simulink model "single_phase_dab"  (R2026b)
settings: Solver=ode23tb  StopTime=param.sim.simlength  FixedStep=param.glb_time.tc  MaxStep=param.glb_time.tc
values from neighbouring files (symbols this model uses):
  param = struct()    [init_model.m]
libraries: fl_lib x22, nesl_utility x15, discrete_time_low_pass_filter x7, lithium_ion_battery x2, pi_ctrl x2, full_bridge_ideal_switch x2, full_bridge_mosfet_based_with_thermal_model x2, full_bridge_mosfet_based_with_thermal_model_zvs x2, dab_single_phase_pwm_modulator x1, single_phase_transformer x1
(part 1 of 2)
settings Model: Creator=LTNBDA  LastModifiedBy=d.bagnara
settings SolverCC: AutoInsertRateTranBlk=on  SolverResetMethod=Robust  ZeroCrossAlgorithm=Adaptive  ZeroCrossControl=EnableAll
settings DataIOCC: DSMLogging=off  LimitDataPoints=on  MaxDataPoints=1  ReturnWorkspaceOutputs=off  SaveFormat=Array  SaveOutput=off  SaveTime=off  SignalLogging=off  SignalLoggingSaveFormat=ModelDataLogs
settings OptimizationCC: EfficientMapNaN2IntZero=off  LifeSpan=inf  MemsetInitFltsAndDblsToZero=off
settings DebuggingCC: ArithmeticOperatorsInVariantConditions=warning  FcnCallInpInsideContextMsg=warning  MergeDetectMultiDrivingBlocksExec=none  MultiTaskCondExecSysMsg=none  MultiTaskDSMMsg=warning  MultiTaskRateTransMsg=warning  SFNoUnconditionalDefaultTransitionDiag=warning  SFUnexpectedBacktrackingDiag=warning  SaveWithParameterizedLinksMsg=none  SignalResolutionControl=TryResolveAllWithWarning  SolverPrmCheckMsg=warning  StateNameClashWarn=warning
settings HardwareCC: ProdEndianess=Unspecified  ProdEqTarget=off  ProdHWDeviceType=Generic->64-bit Embedded Processor (LP64)  ProdIntDivRoundTo=Undefined  ProdLargestAtomicFloat=None  TargetEndianess=LittleEndian  TargetHWDeviceType=MATLAB Host  TargetIntDivRoundTo=Zero  TargetLongLongMode=on
settings ModelReferenceCC: PropagateSignalLabelsOutOfModel=off
settings SFSimCC: CustomCodeUndefinedFunction=UseInterfaceOnly  SimUseLocalCustomCode=off
settings SFSimCC: SimCustomHeaderCode=|
  | #include "rpi.h"
  | #include "rpi_simulink.h"
  | #include "mavgflt.h"
  | #include "mavgflt_simulink.h"
  | #include "mavgflts.h"
  | #include "mavgflts_simulink.h"
  | #include "dsmavgflt.h"
  | #include "dsmavgflt_simulink.h"
  | #include "bemf_obsv.h"
  | #include "bemf_obsv_simulink.h"
  | #include "bemf_obsv_load_est.h"
  | #include "bemf_obsv_load_est_simulink.h"
  | #include "dqvector_pi.h"
  | #include "dqvector_pi_simulink.h"
  | #include "sv_pwm_simulink.h"
  | #include "sv_pwm.h"
  | #include "first_harmonic_tracker.h"
  | #include "first_harmonic_tracker_simulink.h"
  | #include "dqpll_thyr.h"
  | #include "dqpll_thyr_simulink.h"
  | #include "dqpll_grid.h"
  | #include "dqpll_grid_simulink.h"
  | #include "linear_double_integrator_observer_simulink.h"
  | #include "linear_double_integrator_observer.h"
  | #include "sv_pwm_cm_simulink.h"
  | #include "sv_pwm_cm.h"
settings SFSimCC: SimUserIncludeDirs=|
  | include
  | src
settings SFSimCC: SimUserSources=|
  | "rpi.c"
  | "rpi_simulink.c"
  | "mavgflt_simulink.c"
  | "mavgflt.c"
  | "mavgflts_simulink.c"
  | "mavgflts.c"
  | "dsmavgflt_simulink.c"
  | "dsmavgflt.c"
  | "bemf_obsv_simulink.c"
  | "bemf_obsv.c"
  | "bemf_obsv_load_est_simulink.c"
  | "bemf_obsv_load_est.c"
  | "dqvector_pi.c"
  | "dqvector_pi_simulink.c"
  | "sv_pwm_simulink.c"
  | "sv_pwm.c"
  | "first_harmonic_tracker_simulink.c"
  | "first_harmonic_tracker.c"
  | "dqpll_thyr_simulink.c"
  | "dqpll_thyr.c"
  | "dqpll_grid_simulink.c"
  | "dqpll_grid.c"
  | "linear_double_integrator_observer_simulink.c"
  | "linear_double_integrator_observer.c"
  | "sv_pwm_cm_simulink.c"
  | "sv_pwm_cm.c"
settings RTWCC: CustomInclude=ccaller  RTWUseLocalCustomCode=off
settings CodeAppCC: StateflowObjectComments=on
settings GRTTargetCC: CombineOutputUpdateFcns=off  GRTInterface=on  TargetLangStandard=C89/C90 (ANSI)
settings ConfigComp: CovExternalEMLEnable=off  CovSaveCumulativeToWorkspaceVar=on  CovSaveSingleToWorkspaceVar=on
settings SimscapeCC: SimscapeNormalizeSystem=off  SimscapeUseEnergyAccounting=off

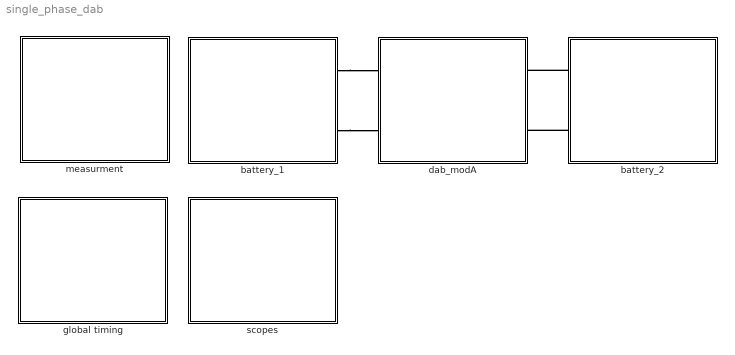
== system single_phase_dab ==
  battery_1 : Subsystem
  battery_2 : Subsystem
  dab_modA : Subsystem
  global timing : Subsystem
  measurment : Subsystem
  scopes : Subsystem
  connections:
  battery_2/RConn2 -- dab_modA/RConn2
  battery_2/RConn1 -- dab_modA/RConn1
  battery_1/RConn1 -- dab_modA/LConn1
  battery_1/RConn2 -- dab_modA/LConn2

== system single_phase_dab/battery_1 ==
  Electrical Reference1 : fl_lib/Electrical/Electrical Elements/Electrical Reference
  Solver Configuration : nesl_utility/Solver Configuration  PhysicalDomain=network_engine_domain  SubClassName=solver  LeftPortType=input  RightPortType=generic  Tones=[]  Harmonics=[]  SimulateNoise=off  Profile=off  UseLocalSampling=off  EnableSwitchedLinearOptims=on  FrequencyDomain=off  UseCCode=off  RelTol=0.001  AbsTol=0.001  MinStep=1e-09  ToWorkspace=off  RevertToSquareIcSolve=off  NumHomotopyIterations=100  PhasorMode=off  PhasorModeNumHarmonics=1  ConsistencySolver=NEWTON_FTOL  CanonicalOrdering=UNORDERED  OptimizeIntermediates=UNOPTIMIZED  MulticoreSolverChoice=BACKWARD_EULER  IndexReductionMethod=DerivativeReplacement  DoDC=off  ResidualTolerance=1e-09  ConsistencyTolSource=GLOBAL  ConsistencyAbsTol=0.001  ConsistencyRelTol=0.001  ConsistencyTolFactor=0.001  UseLocalSolver=on  LocalSolverChoice=NE_BACKWARD_EULER_ADVANCER  ResolveIndetEquations=on  FunctionEvalNumThread=1  LocalSolverSampleTime=param.glb_time.tc  DoFixedCost=on  MaxNonlinIter=param.sim.nonlinear_iterations  MaxModeIter=2  ComputeImpulses=off  ImpulseIterations=2  LinearAlgebra=auto  LinearAlgebraNumThread=0  EquationFormulation=NE_TIME_EF  DelaysMemoryBudget=1024  AutomaticFiltering=on  FilteringTimeConstant=0.001  PartitionStorageMethod=AS_NEEDED  PartitionMemoryBudget=1024  PartitionMethod=BALANCED  MultibodyUseLocalSolver=off  MultibodyLocalSolverChoice=ODE1  MultibodyLocalSolverSampleTime=0.001
  litium ion battery 1 : Scope
      settings: ActiveDisplayYMinimum=-166.63080014270002  ActiveDisplayYMaximum=1499.6922306374129  DataLoggingVariableName=ScopeData3
  litium_ion_battery : lithium_ion_battery/lithium_ion_battery  Q=param.battery.pack_1.Q  number_of_cells=param.battery.pack_1.number_of_cells  E_1=param.battery.pack_1.E_1  E0=param.battery.pack_1.E0  E1=param.battery.pack_1.E1  E2=param.battery.pack_1.E2  E3=param.battery.pack_1.E3  Elog=param.battery.pack_1.Elog  R0=param.battery.pack_1.R0  R1=param.battery.pack_1.R1  C1=param.battery.pack_1.C1  M=param.battery.pack_1.M  alpha=param.battery.pack_1.alpha  soc_init=param.battery.pack_1.soc_init  ts_battery=param.glb_time.ts_dab  q1Kalman=param.battery.pack_1.q1Kalman  q2Kalman=param.battery.pack_1.q2Kalman  q3Kalman=param.battery.pack_1.q3Kalman  rKalman=param.battery.pack_1.rKalman  tc=param.glb_time.tc  enable_white_noise_m=0  battery_voltage_init_m=param.battery.ocv_1
  single_phase_ui_measure : Subsystem
  dc+ : PMIOPort  Side=Right
  dc- : PMIOPort  Port=2  Side=Right
  wires:
  litium_ion_battery/1 -> litium ion battery 1/1
  connections:
  single_phase_ui_measure/LConn2 -- litium_ion_battery/RConn2 -- Electrical Reference1/LConn1 -- Solver Configuration/RConn1
  single_phase_ui_measure/RConn1 -- dc+/RConn1
  litium_ion_battery/RConn1 -- single_phase_ui_measure/LConn1
  dc-/RConn1 -- single_phase_ui_measure/RConn2

== system single_phase_dab/battery_2 ==
  Electrical Reference1 : fl_lib/Electrical/Electrical Elements/Electrical Reference
  litium ion battery 2 : Scope
      settings: ActiveDisplayYMinimum=-4779.68523514888  ActiveDisplayYMaximum=38953.418417165572  DataLoggingVariableName=ScopeData3
  litium_ion_battery : lithium_ion_battery/lithium_ion_battery  Q=param.battery.pack_2.Q  number_of_cells=param.battery.pack_2.number_of_cells  E_1=param.battery.pack_2.E_1  E0=param.battery.pack_2.E0  E1=param.battery.pack_2.E1  E2=param.battery.pack_2.E2  E3=param.battery.pack_2.E3  Elog=param.battery.pack_2.Elog  R0=param.battery.pack_2.R0  R1=param.battery.pack_2.R1  C1=param.battery.pack_2.C1  M=param.battery.pack_2.M  alpha=param.battery.pack_2.alpha  soc_init=param.battery.pack_2.soc_init  ts_battery=param.glb_time.ts_dab  q1Kalman=param.battery.pack_2.q1Kalman  q2Kalman=param.battery.pack_2.q2Kalman  q3Kalman=param.battery.pack_2.q3Kalman  rKalman=param.battery.pack_2.rKalman  tc=param.glb_time.tc  enable_white_noise_m=0  battery_voltage_init_m=param.battery.ocv_2
  single_phase_ui_measure : Subsystem
  dc+ : PMIOPort  Side=Right
  dc- : PMIOPort  Port=2  Side=Right
  wires:
  litium_ion_battery/1 -> litium ion battery 2/1
  connections:
  dc-/RConn1 -- single_phase_ui_measure/RConn2
  litium_ion_battery/RConn1 -- single_phase_ui_measure/LConn1
  single_phase_ui_measure/RConn1 -- dc+/RConn1
  Electrical Reference1/LConn1 -- litium_ion_battery/RConn2 -- single_phase_ui_measure/LConn2

== system single_phase_dab/dab_modA ==
  dab_ctrl : Subsystem
  dcdc_with_galvanic_isolation : Subsystem
  udc(+) : PMIOPort  Side=Right
  udc(-) : PMIOPort  Port=2  Side=Right
  dc+ : PMIOPort  Port=3  Side=Left
  dc- : PMIOPort  Port=4  Side=Left
  wires:
  dab_ctrl/1(gate_commands) -> dcdc_with_galvanic_isolation/1(gate_commands)
  connections:
  udc(+)/RConn1 -- dcdc_with_galvanic_isolation/RConn1
  udc(-)/RConn1 -- dcdc_with_galvanic_isolation/RConn2
  dc-/RConn1 -- dcdc_with_galvanic_isolation/LConn2
  dc+/RConn1 -- dcdc_with_galvanic_isolation/LConn1

== system single_phase_dab/global timing ==
  From9 : From  Commented=on  GotoTag=local_time_corr_llc_mod1
  Unit Delay : UnitDelay  SampleTime=param.glb_time.tc
  time_afe1 : Subsystem  mask{k=1}
      mask prompts: k "Time Gain"
      mask Display:
      | disp('time-gen');
      | port_label('input', 1, 'crt');
      | port_label('output', 1, 'tout');
  time_afe3 : Subsystem  mask{k=1}
      mask prompts: k "Time Gain"
      mask Display:
      | disp('time-gen');
      | port_label('output', 1, 'tout');
  tag scope: time_dab_module_1=global, time_master=global
  wires:
  time_afe1/1(Out1) -> [time_dab_module_1]
  time_afe3/1(Out1) -> [time_master]
  From9/1 -> Unit Delay/1
  Unit Delay/1 -> time_afe1/1(correction_time)

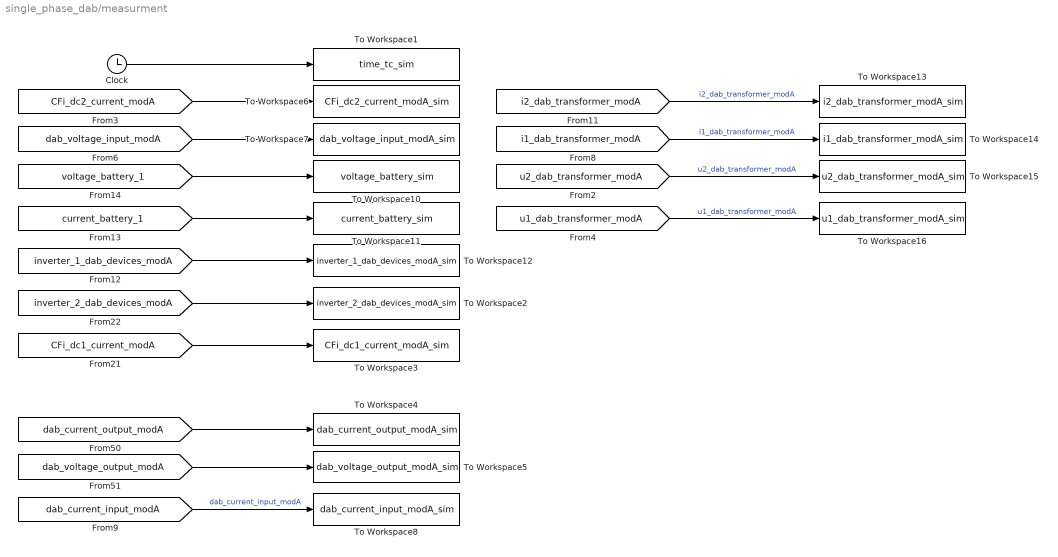
== system single_phase_dab/measurment ==
  Clock : Clock
  To Workspace1 : ToWorkspace  VariableName=time_tc_sim  SampleTime=param.glb_time.tc
      settings: MaxDataPoints=param.glb_time.Nc  Decimation=param.glb_time.decimation_tc
  To Workspace10 : ToWorkspace  VariableName=voltage_battery_sim  SampleTime=param.glb_time.tc
      settings: MaxDataPoints=param.glb_time.Nc  Decimation=param.glb_time.decimation_tc
  To Workspace11 : ToWorkspace  VariableName=current_battery_sim  SampleTime=param.glb_time.tc
      settings: MaxDataPoints=param.glb_time.Nc  Decimation=param.glb_time.decimation_tc
  To Workspace12 : ToWorkspace  VariableName=inverter_1_dab_devices_modA_sim  SampleTime=param.glb_time.tc
      settings: MaxDataPoints=param.glb_time.Nc  Decimation=param.glb_time.decimation_tc
  To Workspace13 : ToWorkspace  VariableName=i2_dab_transformer_modA_sim  SampleTime=param.glb_time.tc
      settings: MaxDataPoints=param.glb_time.Nc  Decimation=param.glb_time.decimation_tc
  To Workspace14 : ToWorkspace  VariableName=i1_dab_transformer_modA_sim  SampleTime=param.glb_time.tc
      settings: MaxDataPoints=param.glb_time.Nc  Decimation=param.glb_time.decimation_tc
  To Workspace15 : ToWorkspace  VariableName=u2_dab_transformer_modA_sim  SampleTime=param.glb_time.tc
      settings: MaxDataPoints=param.glb_time.Nc  Decimation=param.glb_time.decimation_tc
  To Workspace16 : ToWorkspace  VariableName=u1_dab_transformer_modA_sim  SampleTime=param.glb_time.tc
      settings: MaxDataPoints=param.glb_time.Nc  Decimation=param.glb_time.decimation_tc
  To Workspace2 : ToWorkspace  VariableName=inverter_2_dab_devices_modA_sim  SampleTime=param.glb_time.tc
      settings: MaxDataPoints=param.glb_time.Nc  Decimation=param.glb_time.decimation_tc
  To Workspace3 : ToWorkspace  VariableName=CFi_dc1_current_modA_sim  SampleTime=param.glb_time.tc
      settings: MaxDataPoints=param.glb_time.Nc  Decimation=param.glb_time.decimation_tc
  To Workspace4 : ToWorkspace  VariableName=dab_current_output_modA_sim  SampleTime=param.glb_time.tc
      settings: MaxDataPoints=param.glb_time.Nc  Decimation=param.glb_time.decimation_tc
  To Workspace5 : ToWorkspace  VariableName=dab_voltage_output_modA_sim  SampleTime=param.glb_time.tc
      settings: MaxDataPoints=param.glb_time.Nc  Decimation=param.glb_time.decimation_tc
  To Workspace6 : ToWorkspace  VariableName=CFi_dc2_current_modA_sim  SampleTime=param.glb_time.tc
      settings: MaxDataPoints=param.glb_time.Nc  Decimation=param.glb_time.decimation_tc
  To Workspace7 : ToWorkspace  VariableName=dab_voltage_input_modA_sim  SampleTime=param.glb_time.tc
      settings: MaxDataPoints=param.glb_time.Nc  Decimation=param.glb_time.decimation_tc
  To Workspace8 : ToWorkspace  VariableName=dab_current_input_modA_sim  SampleTime=param.glb_time.tc
      settings: MaxDataPoints=param.glb_time.Nc  Decimation=param.glb_time.decimation_tc
  wires:
  Clock/1 -> To Workspace1/1
  [CFi_dc2_current_modA] -> To Workspace6/1
  [dab_voltage_input_modA] -> To Workspace7/1
  [voltage_battery_1] -> To Workspace10/1
  [current_battery_1] -> To Workspace11/1
  [CFi_dc1_current_modA] -> To Workspace3/1
  [dab_voltage_output_modA] -> To Workspace5/1
  [dab_current_output_modA] -> To Workspace4/1
  [inverter_1_dab_devices_modA] -> To Workspace12/1
  [inverter_2_dab_devices_modA] -> To Workspace2/1
  [dab_current_input_modA] -> To Workspace8/1  "dab_current_input_modA"
  [i2_dab_transformer_modA] -> To Workspace13/1  "i2_dab_transformer_modA"
  [i1_dab_transformer_modA] -> To Workspace14/1  "i1_dab_transformer_modA"
  [u2_dab_transformer_modA] -> To Workspace15/1  "u2_dab_transformer_modA"
  [u1_dab_transformer_modA] -> To Workspace16/1  "u1_dab_transformer_modA"

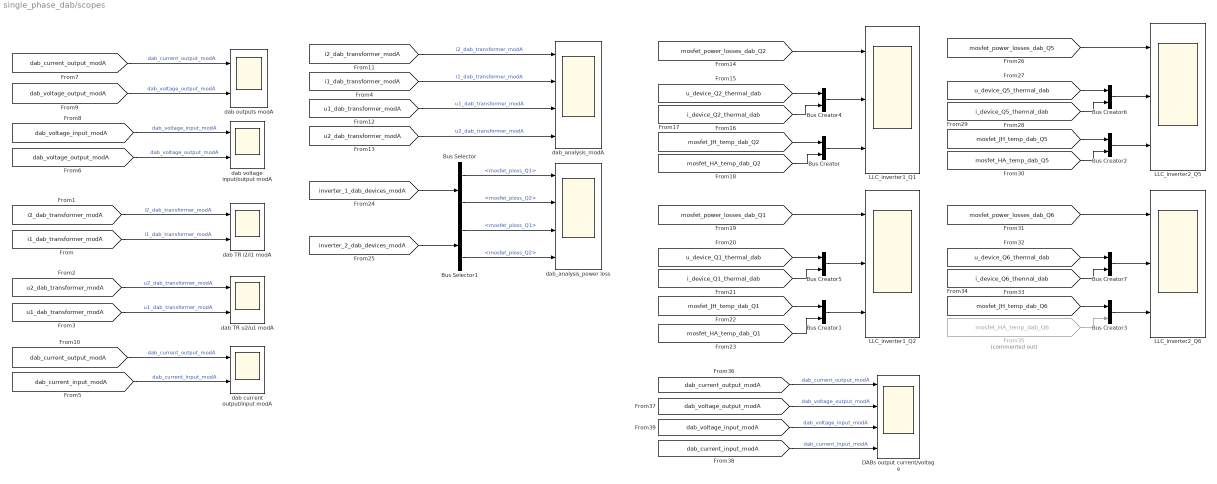
== system single_phase_dab/scopes ==
  Bus Creator{,1..7} (8 alike) : BusCreator  Inputs=2
  Bus Selector : BusSelector  OutputSignals=mosfet_ploss_Q1,mosfet_ploss_Q2
  Bus Selector1 : BusSelector  OutputSignals=mosfet_ploss_Q1,mosfet_ploss_Q2
  DABs output current/voltage : Scope  NumInputPorts=4
      settings: ActiveDisplayString=3  ActiveDisplayYMinimum=1041.3336241461893  ActiveDisplayYMaximum=1127.4737653725774  DataLoggingVariableName=ScopeData9
  From35 : From  Commented=on  GotoTag=mosfet_HA_temp_dab_Q6
  LLC_inverter1_Q1 : Scope  NumInputPorts=3
      settings: SampleTime=param.glb_time.tc  ActiveDisplayYMinimum=-11.051389323298961  ActiveDisplayYMaximum=99.462503909690668
  LLC_inverter1_Q2 : Scope  NumInputPorts=3
      settings: SampleTime=param.glb_time.tc  ActiveDisplayYMinimum=-34.225852820065704  ActiveDisplayYMaximum=308.0326753805914  DataLoggingVariableName=ScopeData5
  LLC_inverter2_Q5 : Scope  NumInputPorts=3
      settings: SampleTime=param.glb_time.tc  ActiveDisplayYMinimum=-28.874053400724897  ActiveDisplayYMaximum=276.48281575164191  DataLoggingVariableName=ScopeData7
  LLC_inverter2_Q6 : Scope  NumInputPorts=3
      settings: SampleTime=param.glb_time.tc  ActiveDisplayYMinimum=-64.618426980891613  ActiveDisplayYMaximum=628.02605861789084  DataLoggingVariableName=ScopeData11
  dab TR i2/i1 modA : Scope  NumInputPorts=2
      settings: SampleTime=param.glb_time.tc  ActiveDisplayYMinimum=-635.40775093889511  ActiveDisplayYMaximum=640.17928955383354  DataLoggingVariableName=ScopeData13
  dab TR u2/u1 modA : Scope  NumInputPorts=2
      settings: SampleTime=param.glb_time.tc  ActiveDisplayYMinimum=-893.62031856834165  ActiveDisplayYMaximum=653.92363611228757  DataLoggingVariableName=ScopeData4
  dab current output/input modA : Scope  NumInputPorts=2
      settings: SampleTime=param.glb_time.tc  ActiveDisplayYMinimum=-767.63883399030738  ActiveDisplayYMaximum=849.74730240031818  DataLoggingVariableName=ScopeData8
  dab outputs modA : Scope  NumInputPorts=2
      settings: SampleTime=param.glb_time.tc  ActiveDisplayYMinimum=-607.9269366315915  ActiveDisplayYMaximum=560.81637051145344  DataLoggingVariableName=ScopeData6
  dab voltage input/output modA : Scope  NumInputPorts=2
      settings: SampleTime=param.glb_time.tc  ActiveDisplayYMinimum=1118.1896415738145  ActiveDisplayYMaximum=1466.7276256846569  DataLoggingVariableName=ScopeData10
  dab_analysis_modA : Scope  NumInputPorts=4
      settings: SampleTime=param.glb_time.tc  ActiveDisplayYMinimum=-1439.3094144547488  ActiveDisplayYMaximum=1439.3301053904904  DataLoggingVariableName=ScopeData15
  dab_analysis_power loss : Scope  NumInputPorts=4
      settings: SampleTime=param.glb_time.tc  ActiveDisplayYMinimum=-29.123739079352042  ActiveDisplayYMaximum=278.761470949118  DataLoggingVariableName=ScopeData17
  wires:
  [mosfet_power_losses_dab_Q6] -> LLC_inverter2_Q6/1
  [inverter_1_dab_devices_modA] -> Bus Selector/1
  [u_device_Q5_thermal_dab] -> Bus Creator6/1
  [u_device_Q2_thermal_dab] -> Bus Creator4/1
  [mosfet_JH_temp_dab_Q6] -> Bus Creator3/1
  [u2_dab_transformer_modA] -> dab TR u2/u1 modA/1  "u2_dab_transformer_modA"
  [mosfet_JH_temp_dab_Q1] -> Bus Creator1/1
  [mosfet_power_losses_dab_Q1] -> LLC_inverter1_Q2/1
  [mosfet_power_losses_dab_Q2] -> LLC_inverter1_Q1/1
  [i_device_Q6_thermal_dab] -> Bus Creator7/2
  [i1_dab_transformer_modA] -> dab_analysis_modA/2  "i1_dab_transformer_modA"
  [i_device_Q5_thermal_dab] -> Bus Creator6/2
  [mosfet_JH_temp_dab_Q2] -> Bus Creator/1
  Bus Creator1/1 -> LLC_inverter1_Q2/3
  [mosfet_power_losses_dab_Q5] -> LLC_inverter2_Q5/1
  [dab_current_output_modA] -> dab current output/input modA/1  "dab_current_output_modA"
  [i_device_Q2_thermal_dab] -> Bus Creator4/2
  [dab_current_input_modA] -> dab current output/input modA/2  "dab_current_input_modA"
  [dab_voltage_output_modA] -> dab outputs modA/2  "dab_voltage_output_modA"
  [mosfet_HA_temp_dab_Q5] -> Bus Creator2/2
  Bus Creator4/1 -> LLC_inverter1_Q1/2
  [dab_current_output_modA] -> dab outputs modA/1  "dab_current_output_modA"
  [i2_dab_transformer_modA] -> dab_analysis_modA/1  "i2_dab_transformer_modA"
  [dab_voltage_output_modA] -> DABs output current/voltage/2  "dab_voltage_output_modA"
  Bus Creator5/1 -> LLC_inverter1_Q2/2
  [u1_dab_transformer_modA] -> dab_analysis_modA/3  "u1_dab_transformer_modA"
  [mosfet_HA_temp_dab_Q1] -> Bus Creator1/2
  [dab_voltage_output_modA] -> dab voltage input/output modA/2  "dab_voltage_output_modA"
  [mosfet_JH_temp_dab_Q5] -> Bus Creator2/1
  Bus Selector/1 -> dab_analysis_power loss/1  "<mosfet_ploss_Q1>"
  [u_device_Q6_thermal_dab] -> Bus Creator7/1
  [i1_dab_transformer_modA] -> dab TR i2/i1 modA/2  "i1_dab_transformer_modA"
  Bus Creator2/1 -> LLC_inverter2_Q5/3
  [i_device_Q1_thermal_dab] -> Bus Creator5/2
  [mosfet_HA_temp_dab_Q2] -> Bus Creator/2
  [dab_current_input_modA] -> DABs output current/voltage/4  "dab_current_input_modA"
  Bus Creator/1 -> LLC_inverter1_Q1/3
  [i2_dab_transformer_modA] -> dab TR i2/i1 modA/1  "i2_dab_transformer_modA"
  Bus Selector/2 -> dab_analysis_power loss/2  "<mosfet_ploss_Q2>"
  [dab_voltage_input_modA] -> dab voltage input/output modA/1  "dab_voltage_input_modA"
  [inverter_2_dab_devices_modA] -> Bus Selector1/1
  [u1_dab_transformer_modA] -> dab TR u2/u1 modA/2  "u1_dab_transformer_modA"
  Bus Selector1/2 -> dab_analysis_power loss/4  "<mosfet_ploss_Q2>"
  Bus Creator7/1 -> LLC_inverter2_Q6/2
  [u2_dab_transformer_modA] -> dab_analysis_modA/4  "u2_dab_transformer_modA"
  [u_device_Q1_thermal_dab] -> Bus Creator5/1
  Bus Creator6/1 -> LLC_inverter2_Q5/2
  Bus Selector1/1 -> dab_analysis_power loss/3  "<mosfet_ploss_Q1>"
  [dab_voltage_input_modA] -> DABs output current/voltage/3  "dab_voltage_input_modA"
  [dab_current_output_modA] -> DABs output current/voltage/1  "dab_current_output_modA"
  From35/1 -> Bus Creator3/2
  Bus Creator3/1 -> LLC_inverter2_Q6/3

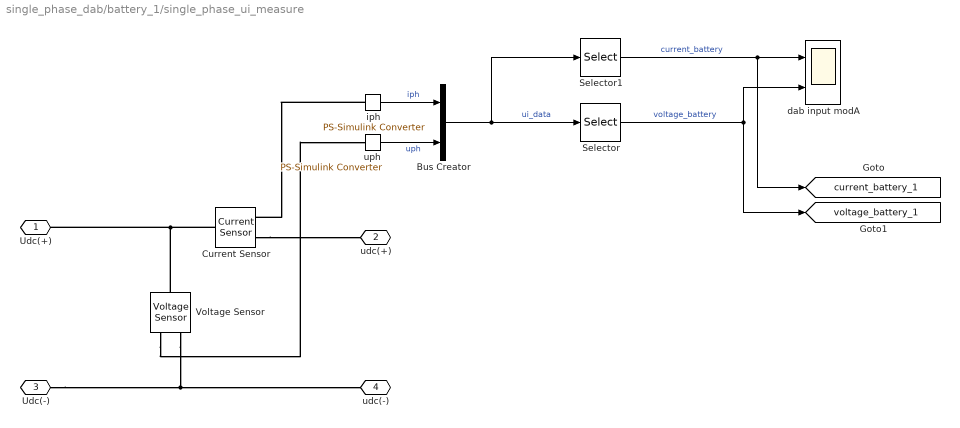
== system single_phase_dab/battery_1/single_phase_ui_measure ==
  Bus Creator : BusCreator  Inputs=2
  Current Sensor : fl_lib/Electrical/Electrical Sensors/Current Sensor
  Selector : Selector  InputPortWidth=2  IndexOptions=Index vector (dialog)  Indices=2  OutputSizes=1  RuntimeRangeChecks=off
  Selector1 : Selector  InputPortWidth=2  IndexOptions=Index vector (dialog)  Indices=1  OutputSizes=1  RuntimeRangeChecks=off
  Voltage Sensor : fl_lib/Electrical/Electrical Sensors/Voltage Sensor
  dab input modA : Scope  NumInputPorts=2
      settings: SampleTime=param.glb_time.tc  ActiveDisplayYMinimum=-4428.9106738971032  ActiveDisplayYMaximum=4853.7975894934307  DataLoggingVariableName=ScopeData2
  iph : nesl_utility/PS-Simulink Converter  PhysicalDomain=network_engine_domain  SubClassName=ps_output  LeftPortType=input  RightPortType=output  PseudoPeriodic=off  Frequencies=[]  VectorFormat=1-D array  Unit=A  AffineConversion=off
  uph : nesl_utility/PS-Simulink Converter  PhysicalDomain=network_engine_domain  SubClassName=ps_output  LeftPortType=input  RightPortType=output  PseudoPeriodic=off  Frequencies=[]  VectorFormat=1-D array  Unit=V  AffineConversion=off
  Udc(+) : PMIOPort  Side=Left
  udc(+) : PMIOPort  Port=2  Side=Right
  Udc(-) : PMIOPort  Port=3  Side=Left
  udc(-) : PMIOPort  Port=4  Side=Right
  tag scope: current_battery_1=global, voltage_battery_1=global
  wires:
  Bus Creator/1 -> Selector/1, Selector1/1  "ui_data"
  iph/1 -> Bus Creator/1  "iph"
  uph/1 -> Bus Creator/2  "uph"
  Selector1/1 -> [current_battery_1], dab input modA/1  "current_battery"
  Selector/1 -> dab input modA/2, [voltage_battery_1]  "voltage_battery"
  connections:
  iph/LConn1 -- Current Sensor/RConn1
  Voltage Sensor/LConn1 -- Current Sensor/LConn1 -- Udc(+)/RConn1
  Current Sensor/RConn2 -- udc(+)/RConn1
  Voltage Sensor/RConn1 -- uph/LConn1
  Voltage Sensor/RConn2 -- Udc(-)/RConn1 -- udc(-)/RConn1

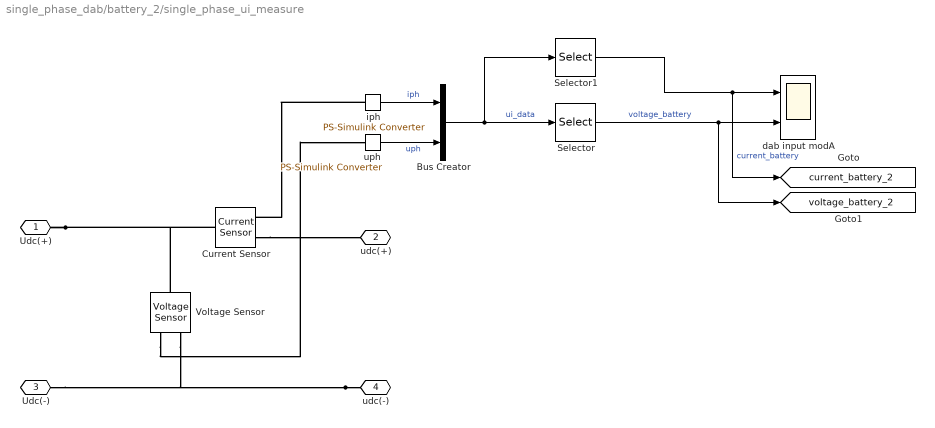
== system single_phase_dab/battery_2/single_phase_ui_measure ==
  Bus Creator : BusCreator  Inputs=2
  Current Sensor : fl_lib/Electrical/Electrical Sensors/Current Sensor
  Selector : Selector  InputPortWidth=2  IndexOptions=Index vector (dialog)  Indices=2  OutputSizes=1  RuntimeRangeChecks=off
  Selector1 : Selector  InputPortWidth=2  IndexOptions=Index vector (dialog)  Indices=1  OutputSizes=1  RuntimeRangeChecks=off
  Voltage Sensor : fl_lib/Electrical/Electrical Sensors/Voltage Sensor
  dab input modA : Scope  NumInputPorts=2
      settings: SampleTime=param.glb_time.tc  ActiveDisplayYMinimum=-363.9315036867377  ActiveDisplayYMaximum=456.02820990604641  DataLoggingVariableName=ScopeData2
  iph : nesl_utility/PS-Simulink Converter  PhysicalDomain=network_engine_domain  SubClassName=ps_output  LeftPortType=input  RightPortType=output  PseudoPeriodic=off  Frequencies=[]  VectorFormat=1-D array  Unit=A  AffineConversion=off
  uph : nesl_utility/PS-Simulink Converter  PhysicalDomain=network_engine_domain  SubClassName=ps_output  LeftPortType=input  RightPortType=output  PseudoPeriodic=off  Frequencies=[]  VectorFormat=1-D array  Unit=V  AffineConversion=off
  Udc(+) : PMIOPort  Side=Left
  udc(+) : PMIOPort  Port=2  Side=Right
  Udc(-) : PMIOPort  Port=3  Side=Left
  udc(-) : PMIOPort  Port=4  Side=Right
  tag scope: current_battery_2=global, voltage_battery_2=global
  wires:
  Selector/1 -> [voltage_battery_2], dab input modA/2  "voltage_battery"
  Selector1/1 -> dab input modA/1, [current_battery_2]  "current_battery"
  uph/1 -> Bus Creator/2  "uph"
  iph/1 -> Bus Creator/1  "iph"
  Bus Creator/1 -> Selector1/1, Selector/1  "ui_data"
  connections:
  udc(-)/RConn1 -- Udc(-)/RConn1 -- Voltage Sensor/RConn2
  Voltage Sensor/RConn1 -- uph/LConn1
  Current Sensor/RConn2 -- udc(+)/RConn1
  Udc(+)/RConn1 -- Current Sensor/LConn1 -- Voltage Sensor/LConn1
  iph/LConn1 -- Current Sensor/RConn1

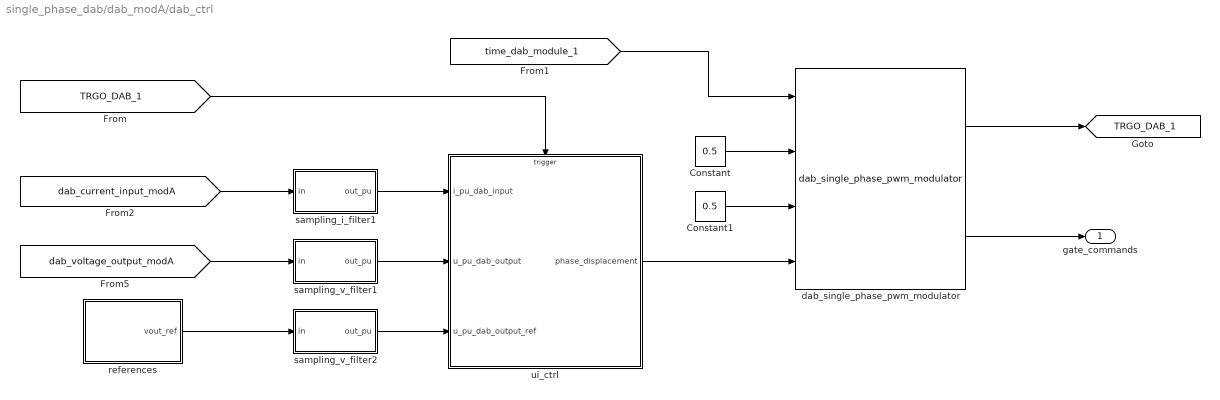
== system single_phase_dab/dab_modA/dab_ctrl ==
  Constant : Constant  Value=0.5
  Constant1 : Constant  Value=0.5
  dab_single_phase_pwm_modulator : dab_single_phase_pwm_modulator/dab_single_phase_pwm_modulator  fPWM_DAB=param.glb_time.fPWM_DAB  m_up=1  m_low=0  dead_time_DAB=param.glb_time.dead_time_DAB  pos_cmd_gate=18  neg_cmd_gate=-3  polarity=-1  tc=param.glb_time.tc  max_phase_displacement=param.dab.mod.phi_max  trgo_double_update=param.glb_time.TRGO_DAB_double_update
  references : Subsystem
  sampling_i_filter1 : Subsystem
  sampling_v_filter1 : Subsystem
  sampling_v_filter2 : Subsystem
  ui_ctrl : Subsystem
  gate_commands : Outport
  tag scope: TRGO_DAB_1=global
  wires:
  [dab_voltage_output_modA] -> sampling_v_filter1/1(in)
  [dab_current_input_modA] -> sampling_i_filter1/1(in)
  sampling_i_filter1/1(out_pu) -> ui_ctrl/1(i_pu_dab_input)
  sampling_v_filter1/1(out_pu) -> ui_ctrl/2(u_pu_dab_output)
  sampling_v_filter2/1(out_pu) -> ui_ctrl/3(u_pu_dab_output_ref)
  references/1(vout_ref) -> sampling_v_filter2/1(in)
  dab_single_phase_pwm_modulator/2 -> gate_commands/1
  [time_dab_module_1] -> dab_single_phase_pwm_modulator/1
  dab_single_phase_pwm_modulator/1 -> [TRGO_DAB_1]
  [TRGO_DAB_1] -> ui_ctrl/Trigger
  Constant/1 -> dab_single_phase_pwm_modulator/2
  Constant1/1 -> dab_single_phase_pwm_modulator/3
  ui_ctrl/1(phase_displacement) -> dab_single_phase_pwm_modulator/4

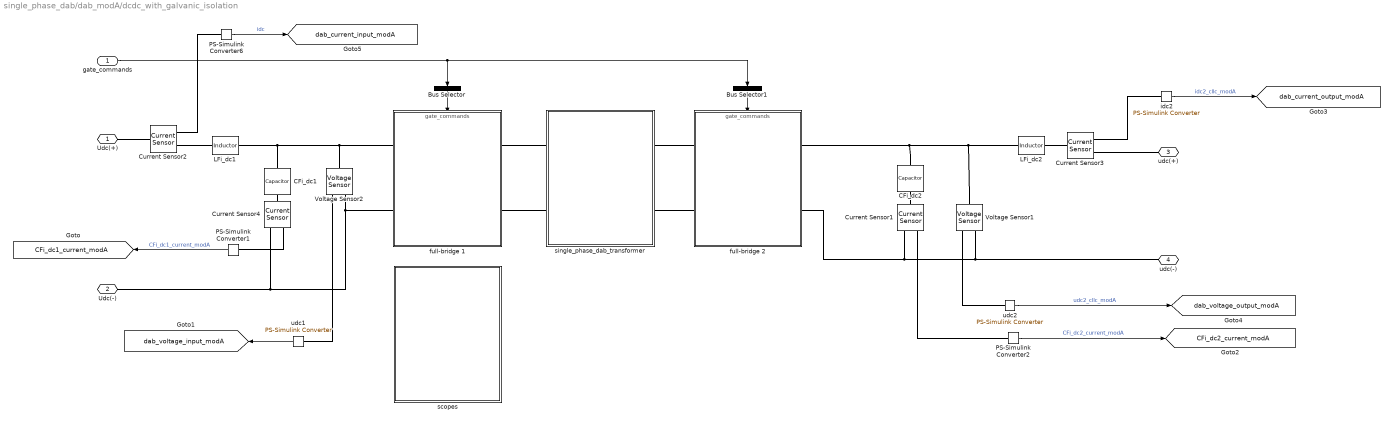
== system single_phase_dab/dab_modA/dcdc_with_galvanic_isolation ==
  gate_commands : Inport
  Bus Selector : BusSelector  OutputSignals=full_bridge1.gate_cmd_Q1,full_bridge1.gate_cmd_Q2,full_bridge1.gate_cmd_Q3,full_bridge1.gate_cmd_Q4  OutputAsBus=on
  Bus Selector1 : BusSelector  OutputSignals=full_bridge2.gate_cmd_Q1,full_bridge2.gate_cmd_Q2,full_bridge2.gate_cmd_Q3,full_bridge2.gate_cmd_Q4  OutputAsBus=on
  CFi_dc1 : fl_lib/Electrical/Electrical Elements/Capacitor  c=param.dab.hw.Cdc_dc1 F  r=param.dab.hw.RCdc_dc1 Ohm  g=0 1/Ohm  i_specify=off  i_priority=None  i=0 A  i_nominal_specify=off  i_nominal_value=1  i_nominal_unit=A  v_specify=off  v_priority=None  v=0 V  v_nominal_specify=off  v_nominal_value=1  v_nominal_unit=V  vc_specify=on  vc_priority=High  vc=param.dab.ic.vc_dc1 V  vc_nominal_specify=off  vc_nominal_value=1  vc_nominal_unit=V
  CFi_dc2 : fl_lib/Electrical/Electrical Elements/Capacitor  c=param.dab.hw.Cdc_dc2 F  r=param.dab.hw.RCdc_dc2 Ohm  g=0 1/Ohm  i_specify=off  i_priority=None  i=0 A  i_nominal_specify=off  i_nominal_value=1  i_nominal_unit=A  v_specify=off  v_priority=None  v=0 V  v_nominal_specify=off  v_nominal_value=1  v_nominal_unit=V  vc_specify=on  vc_priority=High  vc=param.dab.ic.vc_dc2 V  vc_nominal_specify=off  vc_nominal_value=1  vc_nominal_unit=V
  Current Sensor{1..4} (4 alike) : fl_lib/Electrical/Electrical Sensors/Current Sensor
  LFi_dc1 : fl_lib/Electrical/Electrical Elements/Inductor  l=param.dab.hw.Ldc_dc1 H  r=param.dab.hw.RLdc_dc1 Ohm  g=1e-9 1/Ohm  i_specify=off  i_priority=None  i=0 A  i_nominal_specify=off  i_nominal_value=1  i_nominal_unit=A  v_specify=off  v_priority=None  v=0 V  v_nominal_specify=off  v_nominal_value=1  v_nominal_unit=V  i_L_specify=off  i_L_priority=High  i_L=0 A  i_L_nominal_specify=off  i_L_nominal_value=1  i_L_nominal_unit=A
  LFi_dc2 : fl_lib/Electrical/Electrical Elements/Inductor  l=param.dab.hw.Ldc_dc2 H  r=param.dab.hw.RLdc_dc2 Ohm  g=1e-9 1/Ohm  i_specify=off  i_priority=None  i=0 A  i_nominal_specify=off  i_nominal_value=1  i_nominal_unit=A  v_specify=off  v_priority=None  v=0 V  v_nominal_specify=off  v_nominal_value=1  v_nominal_unit=V  i_L_specify=off  i_L_priority=High  i_L=0 A  i_L_nominal_specify=off  i_L_nominal_value=1  i_L_nominal_unit=A
  PS-Simulink Converter1 : nesl_utility/PS-Simulink Converter  PhysicalDomain=network_engine_domain  SubClassName=ps_output  LeftPortType=input  RightPortType=output  PseudoPeriodic=off  Frequencies=[]  VectorFormat=1-D array  Unit=A  AffineConversion=on
  PS-Simulink Converter2 : nesl_utility/PS-Simulink Converter  PhysicalDomain=network_engine_domain  SubClassName=ps_output  LeftPortType=input  RightPortType=output  PseudoPeriodic=off  Frequencies=[]  VectorFormat=1-D array  Unit=A  AffineConversion=on
  PS-Simulink Converter6 : nesl_utility/PS-Simulink Converter  PhysicalDomain=network_engine_domain  SubClassName=ps_output  LeftPortType=input  RightPortType=output  PseudoPeriodic=off  Frequencies=[]  VectorFormat=1-D array  Unit=A  AffineConversion=on
  Voltage Sensor1 : fl_lib/Electrical/Electrical Sensors/Voltage Sensor
  Voltage Sensor2 : fl_lib/Electrical/Electrical Sensors/Voltage Sensor
  full-bridge 1 : Subsystem
      settings: PortSchema="{\"entries\":[{\"content\":{\"sides\":[{\"content\":{\"connectorIds\":[\"LConn1\",\"LConn2\"]},\"type\":\"ConnectorPlacement.EquallySpacedRectSide\",\"uuid\":\"c872503a-61af-4937-bdf2-4de4f8645573\"},{\"content\":{\"connectorIds\":[\"RConn1\",\"RConn2\"],\"side\":\"RIGHT\"},\"type\":\"ConnectorPlacement.EquallySpacedRectSide\",\"uuid\":\"3b83f060-86a2-4569-84b5-d9f7c0485347\"},{\"content\":{\"connectorIds\":[\"In1\"],\"side\":\"TOP\"},\"type\":\"ConnectorPlacement.EquallySpacedRectSide\",\"uuid\":\"bf191d46-ce71-4d15-9dd0-24cc57253577\"}]},\"type\":\"ConnectorPlacement.EquallySpacedConnector\",\"uuid\":\"1b28ceee-25d0-45ae-a3c4-c2563f0d63ba\"}],\"packageUris\":[\"http://schema.mathworks.com/mf0/Connector/R2020b\"],\"version\":\"1.0\"}"
  full-bridge 2 : Subsystem
      settings: PortSchema="{\"entries\":[{\"content\":{\"sides\":[{\"content\":{\"connectorIds\":[\"LConn1\",\"LConn2\"]},\"type\":\"ConnectorPlacement.EquallySpacedRectSide\",\"uuid\":\"c872503a-61af-4937-bdf2-4de4f8645573\"},{\"content\":{\"connectorIds\":[\"RConn1\",\"RConn2\"],\"side\":\"RIGHT\"},\"type\":\"ConnectorPlacement.EquallySpacedRectSide\",\"uuid\":\"3b83f060-86a2-4569-84b5-d9f7c0485347\"},{\"content\":{\"connectorIds\":[\"In1\"],\"side\":\"TOP\"},\"type\":\"ConnectorPlacement.EquallySpacedRectSide\",\"uuid\":\"bf191d46-ce71-4d15-9dd0-24cc57253577\"}]},\"type\":\"ConnectorPlacement.EquallySpacedConnector\",\"uuid\":\"1b28ceee-25d0-45ae-a3c4-c2563f0d63ba\"}],\"packageUris\":[\"http://schema.mathworks.com/mf0/Connector/R2020b\"],\"version\":\"1.0\"}"
  idc2 : nesl_utility/PS-Simulink Converter  PhysicalDomain=network_engine_domain  SubClassName=ps_output  LeftPortType=input  RightPortType=output  PseudoPeriodic=off  Frequencies=[]  VectorFormat=1-D array  Unit=A  AffineConversion=off
  scopes : Subsystem
  single_phase_dab_transformer : Subsystem
  udc1 : nesl_utility/PS-Simulink Converter  PhysicalDomain=network_engine_domain  SubClassName=ps_output  LeftPortType=input  RightPortType=output  PseudoPeriodic=off  Frequencies=[]  VectorFormat=1-D array  Unit=V  AffineConversion=off
  udc2 : nesl_utility/PS-Simulink Converter  PhysicalDomain=network_engine_domain  SubClassName=ps_output  LeftPortType=input  RightPortType=output  PseudoPeriodic=off  Frequencies=[]  VectorFormat=1-D array  Unit=V  AffineConversion=off
  Udc(+) : PMIOPort  Side=Left
  Udc(-) : PMIOPort  Port=2  Side=Left
  udc(+) : PMIOPort  Port=3  Side=Right
  udc(-) : PMIOPort  Port=4  Side=Right
  tag scope: CFi_dc1_current_modA=global, CFi_dc2_current_modA=global, dab_current_input_modA=global, dab_current_output_modA=global, dab_voltage_input_modA=global, dab_voltage_output_modA=global
  wires:
  gate_commands/1 -> Bus Selector1/1, Bus Selector/1
  PS-Simulink Converter6/1 -> [dab_current_input_modA]  "idc"
  Bus Selector/1 -> full-bridge 1/1(gate_commands)
  Bus Selector1/1 -> full-bridge 2/1(gate_commands)
  udc2/1 -> [dab_voltage_output_modA]  "udc2_cllc_modA"
  PS-Simulink Converter2/1 -> [CFi_dc2_current_modA]  "CFi_dc2_current_modA"
  idc2/1 -> [dab_current_output_modA]  "idc2_cllc_modA"
  udc1/1 -> [dab_voltage_input_modA]
  PS-Simulink Converter1/1 -> [CFi_dc1_current_modA]  "CFi_dc1_current_modA"
  connections:
  full-bridge 1/LConn2 -- single_phase_dab_transformer/LConn2
  full-bridge 1/RConn1 -- Voltage Sensor2/LConn1 -- CFi_dc1/LConn1 -- LFi_dc1/RConn1
  full-bridge 1/RConn2 -- Voltage Sensor2/RConn2 -- Current Sensor4/RConn2 -- Udc(-)/RConn1
  full-bridge 1/LConn1 -- single_phase_dab_transformer/LConn1
  LFi_dc1/LConn1 -- Current Sensor2/RConn2
  Udc(+)/RConn1 -- Current Sensor2/LConn1
  Current Sensor2/RConn1 -- PS-Simulink Converter6/LConn1
  full-bridge 2/LConn1 -- single_phase_dab_transformer/RConn1
  full-bridge 2/LConn2 -- single_phase_dab_transformer/RConn2
  CFi_dc2/LConn1 -- full-bridge 2/RConn1 -- LFi_dc2/LConn1 -- Voltage Sensor1/LConn1
  udc(-)/RConn1 -- full-bridge 2/RConn2 -- Current Sensor1/RConn2 -- Voltage Sensor1/RConn2
  PS-Simulink Converter2/LConn1 -- Current Sensor1/RConn1
  Current Sensor3/RConn2 -- udc(+)/RConn1
  Voltage Sensor1/RConn1 -- udc2/LConn1
  idc2/LConn1 -- Current Sensor3/RConn1
  LFi_dc2/RConn1 -- Current Sensor3/LConn1
  CFi_dc2/RConn1 -- Current Sensor1/LConn1
  Voltage Sensor2/RConn1 -- udc1/LConn1
  Current Sensor4/LConn1 -- CFi_dc1/RConn1
  Current Sensor4/RConn1 -- PS-Simulink Converter1/LConn1

== system single_phase_dab/global timing/time_afe1 ==
  correction_time : Inport
  Constant : Constant
  Gain : Gain  Gain=k
  Product : Product
  Sum : Sum  Inputs=|++
  time_1 : Clock
  Out1 : Outport
  wires:
  time_1/1 -> Gain/1
  Gain/1 -> Product/1
  Product/1 -> Out1/1
  correction_time/1 -> Sum/1
  Sum/1 -> Product/2
  Constant/1 -> Sum/2

== system single_phase_dab/global timing/time_afe3 ==
  Gain : Gain  Gain=k
  time_1 : Clock
  Out1 : Outport
  wires:
  Gain/1 -> Out1/1
  time_1/1 -> Gain/1

== system single_phase_dab/dab_modA/dab_ctrl/references ==
  Rate Limiter : RateLimiter  RisingSlewLimit=param.dab.hw.udc2_nom*10  FallingSlewLimit=-param.dab.hw.udc2_nom*10  SampleTimeMode=inherited
  Vout_dc_nom : Step  Time=1e-3  FinalValue=param.dab.hw.udc2_nom  SampleTime=0
  vout_ref : Outport
  wires:
  Rate Limiter/1 -> vout_ref/1
  Vout_dc_nom/1 -> Rate Limiter/1

== system single_phase_dab/dab_modA/dab_ctrl/sampling_i_filter1 ==
  in : Inport
  1/Ti3 : Gain  Gain=1/param.dab.hw.Idc_FS  OutDataTypeStr=double  SaturateOnIntegerOverflow=on  ParamDataTypeStr=Inherit: Same as input
  out_pu : Outport
  wires:
  in/1 -> 1/Ti3/1
  1/Ti3/1 -> out_pu/1

== system single_phase_dab/dab_modA/dab_ctrl/sampling_v_filter1 ==
  in : Inport
  1/Ti3 : Gain  Gain=1/param.dab.hw.Vdc_FS  OutDataTypeStr=double  SaturateOnIntegerOverflow=on  ParamDataTypeStr=Inherit: Same as input
  out_pu : Outport
  wires:
  in/1 -> 1/Ti3/1
  1/Ti3/1 -> out_pu/1

== system single_phase_dab/dab_modA/dab_ctrl/sampling_v_filter2 ==
  in : Inport
  1/Ti3 : Gain  Gain=1/param.dab.hw.Vdc_FS  OutDataTypeStr=double  SaturateOnIntegerOverflow=on  ParamDataTypeStr=Inherit: Same as input
  Saturation : Saturate  UpperLimit=1  LowerLimit=0  OutDataTypeStr=double
  out_pu : Outport
  wires:
  in/1 -> 1/Ti3/1
  1/Ti3/1 -> Saturation/1
  Saturation/1 -> out_pu/1

== system single_phase_dab/dab_modA/dab_ctrl/ui_ctrl ==
  i_pu_dab_input : Inport
  u_pu_dab_output : Inport  Port=2
  u_pu_dab_output_ref : Inport  Port=3
  Trigger : TriggerPort  VariantControl=(inherit)  PortDimensions=1
  dab_ctrl : Subsystem
  scopes : Subsystem
  phase_displacement : Outport
  wires:
  i_pu_dab_input/1 -> dab_ctrl/1(i_pu_dab_input)
  u_pu_dab_output/1 -> dab_ctrl/2(u_pu_dab_output)
  u_pu_dab_output_ref/1 -> dab_ctrl/3(u_pu_dab_output_ref)
  dab_ctrl/1(phase_displacement) -> phase_displacement/1

== system single_phase_dab/dab_modA/dcdc_with_galvanic_isolation/full-bridge 1 ==
  gate_commands : Inport
  data_reference : Subsystem
  full-bridge ideal switch based : full_bridge_ideal_switch/full-bridge ideal switch based  Commented=on  Rds_on=param.dab.ideal_switch.Rds_on  Vdon_diode=param.dab.ideal_switch.Vdon_diode  Rdon_diode=param.dab.ideal_switch.Rdon_diode  Csnubber=param.dab.ideal_switch.Csnubber_zvs  Rsnubber=param.dab.ideal_switch.Rsnubber_zvs  Vth=param.dab.ideal_switch.Vth
  full-bridge mosfet based with thermal model : full_bridge_mosfet_based_with_thermal_model/full-bridge mosfet based with thermal model  Commented=on  mass_heatsink_m=param.thermal.heatsink.no_weight  specific_heat_m=param.thermal.heatsink.cp  rth_mosfet_HA_m=param.thermal.heatsink.Rth_mosfet_HA  rth_mosfet_JH_m=param.dab.mosfet.Rth_mosfet_JH  Rds_on_m=param.dab.mosfet.Rds_on  Vth_m=param.dab.mosfet.Vth  Eon_m=param.dab.mosfet.Eon  Eoff_m=param.dab.mosfet.Eoff  Voff_sw_loss_m=param.dab.mosfet.Voff_sw_losses  Ion_sw_loss_m=param.dab.mosfet.Ion_sw_losses  Vdon_diode_m=param.dab.mosfet.Vdon_diode  Rdon_diode_m=param.dab.mosfet.Rds_on  JunctionTermalMass_m=param.dab.mosfet.JunctionTermalMass  Tambient_m=param.thermal.heatsink.Tambient  DThs_init_m=param.thermal.heatsink.DThs_init
  full-bridge_mosfet_based_ with_thermal_model_zvs : full_bridge_mosfet_based_with_thermal_model_zvs/full-bridge_mosfet_based_ with_thermal_model_zvs  mass_heatsink_m=param.thermal.heatsink.no_weight  specific_heat_m=param.thermal.heatsink.cp  rth_mosfet_HA_m=param.thermal.heatsink.Rth_mosfet_HA  rth_mosfet_JH_m=param.dab.mosfet.Rth_mosfet_JH  Rds_on_m=param.dab.mosfet.Rds_on  Vth_m=param.dab.mosfet.Vth  Eon_m=param.dab.mosfet.Eon  Eoff_m=param.dab.mosfet.Eoff  Voff_sw_loss_m=param.dab.mosfet.Voff_sw_losses  Ion_sw_loss_m=param.dab.mosfet.Ion_sw_losses  Vdon_diode_m=param.dab.mosfet.Vdon_diode  Rdon_diode_m=param.dab.mosfet.Rds_on  JunctionTermalMass_m=param.dab.mosfet.JunctionTermalMass  Tambient_m=param.thermal.heatsink.Tambient  DThs_init_m=param.thermal.heatsink.DThs_init  Csnubber_m=param.dab.mosfet.Csnubber_zvs  Rsnubber_m=param.dab.mosfet.Rsnubber_zvs
  uac_1(+) : PMIOPort  Side=Left
  uac_1(-) : PMIOPort  Port=2  Side=Left
  Udc(+) : PMIOPort  Port=3  Side=Right
  Udc(-) : PMIOPort  Port=4  Side=Right
  wires:
  gate_commands/1 -> full-bridge ideal switch based/1, full-bridge mosfet based with thermal model/1, full-bridge_mosfet_based_ with_thermal_model_zvs/1
  full-bridge_mosfet_based_ with_thermal_model_zvs/1 -> data_reference/1(m)
  connections:
  full-bridge mosfet based with thermal model/RConn1 -- full-bridge ideal switch based/RConn1 -- uac_1(+)/RConn1 -- full-bridge_mosfet_based_ with_thermal_model_zvs/RConn1
  full-bridge mosfet based with thermal model/RConn2 -- full-bridge ideal switch based/RConn2 -- uac_1(-)/RConn1 -- full-bridge_mosfet_based_ with_thermal_model_zvs/RConn2
  Udc(-)/RConn1 -- full-bridge ideal switch based/LConn2 -- full-bridge mosfet based with thermal model/LConn2 -- full-bridge_mosfet_based_ with_thermal_model_zvs/LConn2
  full-bridge mosfet based with thermal model/LConn1 -- full-bridge ideal switch based/LConn1 -- full-bridge_mosfet_based_ with_thermal_model_zvs/LConn1 -- Udc(+)/RConn1

== system single_phase_dab/dab_modA/dcdc_with_galvanic_isolation/full-bridge 2 ==
  gate_commands : Inport
  data_reference : Subsystem
  full-bridge ideal switch based : full_bridge_ideal_switch/full-bridge ideal switch based  Commented=on  Rds_on=param.dab.ideal_switch.Rds_on  Vdon_diode=param.dab.ideal_switch.Vdon_diode  Rdon_diode=param.dab.ideal_switch.Rdon_diode  Csnubber=param.dab.ideal_switch.Csnubber_zvs  Rsnubber=param.dab.ideal_switch.Rsnubber_zvs  Vth=param.dab.ideal_switch.Vth
  full-bridge mosfet based with thermal model : full_bridge_mosfet_based_with_thermal_model/full-bridge mosfet based with thermal model  Commented=on  mass_heatsink_m=param.thermal.heatsink.no_weight  specific_heat_m=param.thermal.heatsink.cp  rth_mosfet_HA_m=param.thermal.heatsink.Rth_mosfet_HA  rth_mosfet_JH_m=param.dab.mosfet.Rth_mosfet_JH  Rds_on_m=param.dab.mosfet.Rds_on  Vth_m=param.dab.mosfet.Vth  Eon_m=param.dab.mosfet.Eon  Eoff_m=param.dab.mosfet.Eoff  Voff_sw_loss_m=param.dab.mosfet.Voff_sw_losses  Ion_sw_loss_m=param.dab.mosfet.Ion_sw_losses  Vdon_diode_m=param.dab.mosfet.Vdon_diode  Rdon_diode_m=param.dab.mosfet.Rds_on  JunctionTermalMass_m=param.dab.mosfet.JunctionTermalMass  Tambient_m=param.thermal.heatsink.Tambient  DThs_init_m=param.thermal.heatsink.DThs_init
  full-bridge_mosfet_based_ with_thermal_model_zvs : full_bridge_mosfet_based_with_thermal_model_zvs/full-bridge_mosfet_based_ with_thermal_model_zvs  mass_heatsink_m=param.thermal.heatsink.no_weight  specific_heat_m=param.thermal.heatsink.cp  rth_mosfet_HA_m=param.thermal.heatsink.Rth_mosfet_HA  rth_mosfet_JH_m=param.dab.mosfet.Rth_mosfet_JH  Rds_on_m=param.dab.mosfet.Rds_on  Vth_m=param.dab.mosfet.Vth  Eon_m=param.dab.mosfet.Eon  Eoff_m=param.dab.mosfet.Eoff  Voff_sw_loss_m=param.dab.mosfet.Voff_sw_losses  Ion_sw_loss_m=param.dab.mosfet.Ion_sw_losses  Vdon_diode_m=param.dab.mosfet.Vdon_diode  Rdon_diode_m=param.dab.mosfet.Rds_on  JunctionTermalMass_m=param.dab.mosfet.JunctionTermalMass  Tambient_m=param.thermal.heatsink.Tambient  DThs_init_m=param.thermal.heatsink.DThs_init  Csnubber_m=param.dab.mosfet.Csnubber_zvs  Rsnubber_m=param.dab.mosfet.Rsnubber_zvs
  uac_2(+) : PMIOPort  Side=Left
  uac_2(-) : PMIOPort  Port=2  Side=Left
  udc(+) : PMIOPort  Port=3  Side=Right
  udc(-) : PMIOPort  Port=4  Side=Right
  wires:
  gate_commands/1 -> full-bridge ideal switch based/1, full-bridge_mosfet_based_ with_thermal_model_zvs/1, full-bridge mosfet based with thermal model/1
  full-bridge_mosfet_based_ with_thermal_model_zvs/1 -> data_reference/1(m)
  connections:
  full-bridge mosfet based with thermal model/RConn1 -- full-bridge ideal switch based/RConn1 -- full-bridge_mosfet_based_ with_thermal_model_zvs/RConn1 -- uac_2(+)/RConn1
  full-bridge mosfet based with thermal model/RConn2 -- full-bridge ideal switch based/RConn2 -- full-bridge_mosfet_based_ with_thermal_model_zvs/RConn2 -- uac_2(-)/RConn1
  full-bridge mosfet based with thermal model/LConn1 -- full-bridge ideal switch based/LConn1 -- full-bridge_mosfet_based_ with_thermal_model_zvs/LConn1 -- udc(+)/RConn1
  full-bridge mosfet based with thermal model/LConn2 -- full-bridge ideal switch based/LConn2 -- full-bridge_mosfet_based_ with_thermal_model_zvs/LConn2 -- udc(-)/RConn1

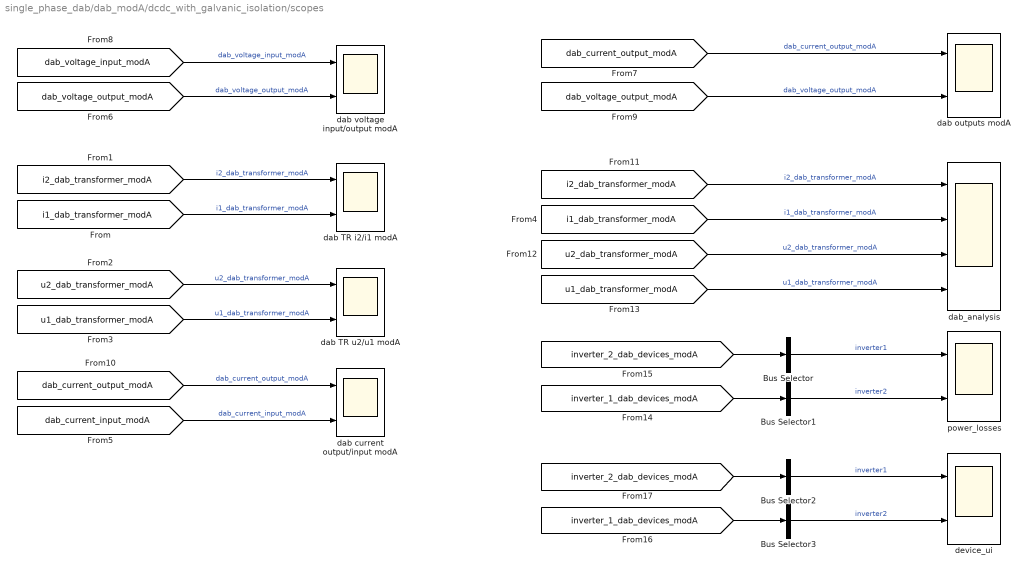
== system single_phase_dab/dab_modA/dcdc_with_galvanic_isolation/scopes ==
  Bus Selector : BusSelector  OutputSignals=mosfet_ploss_Q1,mosfet_ploss_Q2,mosfet_ploss_Q3,mosfet_ploss_Q4  OutputAsBus=on
  Bus Selector1 : BusSelector  OutputSignals=mosfet_ploss_Q1,mosfet_ploss_Q2,mosfet_ploss_Q3,mosfet_ploss_Q4  OutputAsBus=on
  Bus Selector2 : BusSelector  OutputSignals=mosfet_voltage_Q1,mosfet_current_Q1,gate_cmd_Q1,ic_zvs_Q1  OutputAsBus=on
  Bus Selector3 : BusSelector  OutputSignals=mosfet_voltage_Q1,mosfet_current_Q1,gate_cmd_Q1,ic_zvs_Q1  OutputAsBus=on
  dab TR i2/i1 modA : Scope  NumInputPorts=2
      settings: SampleTime=param.glb_time.tc  ActiveDisplayYMinimum=-1133.8385972087863  ActiveDisplayYMaximum=1130.02633442417  DataLoggingVariableName=ScopeData13
  dab TR u2/u1 modA : Scope  NumInputPorts=2
      settings: SampleTime=param.glb_time.tc  ActiveDisplayYMinimum=-1550.0820677220172  ActiveDisplayYMaximum=1550.0802549877285  DataLoggingVariableName=ScopeData4
  dab current output/input modA : Scope  NumInputPorts=2
      settings: SampleTime=param.glb_time.tc  ActiveDisplayYMinimum=-135.33312051034864  ActiveDisplayYMaximum=747.30464050791215  DataLoggingVariableName=ScopeData8
  dab outputs modA : Scope  NumInputPorts=2
      settings: SampleTime=param.glb_time.tc  ActiveDisplayYMinimum=-4075.3303433842134  ActiveDisplayYMaximum=3600.5922239408783  DataLoggingVariableName=ScopeData6
  dab voltage input/output modA : Scope  NumInputPorts=2
      settings: SampleTime=param.glb_time.tc  ActiveDisplayYMinimum=-220.62176138017153  ActiveDisplayYMaximum=1985.59585243125  DataLoggingVariableName=ScopeData10
  dab_analysis : Scope  NumInputPorts=4
      settings: SampleTime=param.glb_time.tc  ActiveDisplayYMinimum=-2638.9202418419895  ActiveDisplayYMaximum=2638.3128773696662  DataLoggingVariableName=ScopeData5
  device_ui : Scope  NumInputPorts=2
      settings: SampleTime=param.glb_time.tc  ActiveDisplayYMinimum=-1039.5583473998261  ActiveDisplayYMaximum=1619.3682765977453  DataLoggingVariableName=ScopeData9
  power_losses : Scope  NumInputPorts=2
      settings: SampleTime=param.glb_time.tc  ActiveDisplayYMinimum=-32.523172649683595  ActiveDisplayYMaximum=292.70855384715242
  wires:
  [dab_voltage_input_modA] -> dab voltage input/output modA/1  "dab_voltage_input_modA"
  [dab_current_output_modA] -> dab current output/input modA/1  "dab_current_output_modA"
  [dab_voltage_output_modA] -> dab voltage input/output modA/2  "dab_voltage_output_modA"
  [dab_current_input_modA] -> dab current output/input modA/2  "dab_current_input_modA"
  [i2_dab_transformer_modA] -> dab TR i2/i1 modA/1  "i2_dab_transformer_modA"
  [i1_dab_transformer_modA] -> dab TR i2/i1 modA/2  "i1_dab_transformer_modA"
  [u2_dab_transformer_modA] -> dab TR u2/u1 modA/1  "u2_dab_transformer_modA"
  [u1_dab_transformer_modA] -> dab TR u2/u1 modA/2  "u1_dab_transformer_modA"
  [dab_voltage_output_modA] -> dab outputs modA/2  "dab_voltage_output_modA"
  [dab_current_output_modA] -> dab outputs modA/1  "dab_current_output_modA"
  [i2_dab_transformer_modA] -> dab_analysis/1  "i2_dab_transformer_modA"
  [i1_dab_transformer_modA] -> dab_analysis/2  "i1_dab_transformer_modA"
  [u2_dab_transformer_modA] -> dab_analysis/3  "u2_dab_transformer_modA"
  [u1_dab_transformer_modA] -> dab_analysis/4  "u1_dab_transformer_modA"
  [inverter_2_dab_devices_modA] -> Bus Selector/1
  Bus Selector/1 -> power_losses/1  "inverter1"
  Bus Selector1/1 -> power_losses/2  "inverter2"
  [inverter_1_dab_devices_modA] -> Bus Selector1/1
  [inverter_1_dab_devices_modA] -> Bus Selector3/1
  Bus Selector3/1 -> device_ui/2  "inverter2"
  Bus Selector2/1 -> device_ui/1  "inverter1"
  [inverter_2_dab_devices_modA] -> Bus Selector2/1

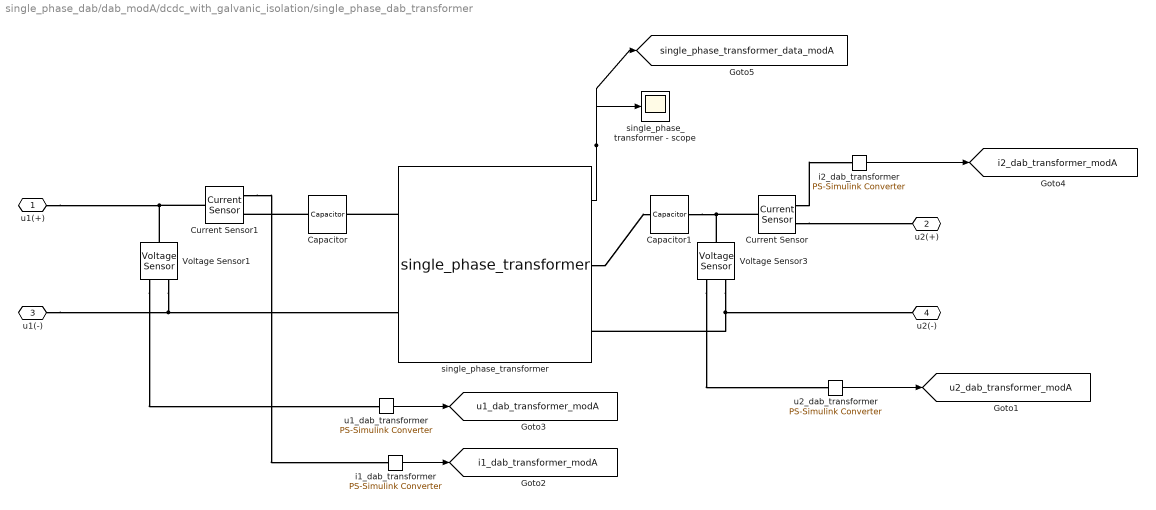
== system single_phase_dab/dab_modA/dcdc_with_galvanic_isolation/single_phase_dab_transformer ==
  Capacitor : fl_lib/Electrical/Electrical Elements/Capacitor  c=param.dab.hw.Cs1 F  r=1e-6 Ohm  g=0 1/Ohm  i_specify=off  i_priority=None  i=0 A  i_nominal_specify=off  i_nominal_value=1  i_nominal_unit=A  v_specify=off  v_priority=None  v=0 V  v_nominal_specify=off  v_nominal_value=1  v_nominal_unit=V  vc_specify=off  vc_priority=High  vc=0 V  vc_nominal_specify=off  vc_nominal_value=1  vc_nominal_unit=V
  Capacitor1 : fl_lib/Electrical/Electrical Elements/Capacitor  c=param.dab.hw.Cs2 F  r=1e-6 Ohm  g=0 1/Ohm  i_specify=off  i_priority=None  i=0 A  i_nominal_specify=off  i_nominal_value=1  i_nominal_unit=A  v_specify=off  v_priority=None  v=0 V  v_nominal_specify=off  v_nominal_value=1  v_nominal_unit=V  vc_specify=off  vc_priority=High  vc=0 V  vc_nominal_specify=off  vc_nominal_value=1  vc_nominal_unit=V
  Current Sensor : fl_lib/Electrical/Electrical Sensors/Current Sensor
  Current Sensor1 : fl_lib/Electrical/Electrical Sensors/Current Sensor
  Voltage Sensor1 : fl_lib/Electrical/Electrical Sensors/Voltage Sensor
  Voltage Sensor3 : fl_lib/Electrical/Electrical Sensors/Voltage Sensor
  i1_dab_transformer : nesl_utility/PS-Simulink Converter  PhysicalDomain=network_engine_domain  SubClassName=ps_output  LeftPortType=input  RightPortType=output  PseudoPeriodic=off  Frequencies=[]  VectorFormat=1-D array  Unit=A  AffineConversion=off
  i2_dab_transformer : nesl_utility/PS-Simulink Converter  PhysicalDomain=network_engine_domain  SubClassName=ps_output  LeftPortType=input  RightPortType=output  PseudoPeriodic=off  Frequencies=[]  VectorFormat=1-D array  Unit=A  AffineConversion=off
  single_phase_transformer : single_phase_transformer/single_phase_transformer  lm_trafo=param.dab.hw.Lm  m1=param.dab.hw.n1  m2=param.dab.hw.n2  rd1_trafo=param.dab.hw.Rs1  rd2_trafo=param.dab.hw.Rs2  ld1_trafo=param.dab.hw.Ld1  ld2_trafo=param.dab.hw.Ld2  rfe_trafo=param.dab.hw.Rfe  length_core=param.dab.hw.core_length  mu0=1.256637e-6  mur=param.dab.hw.core_mur
  single_phase_transformer - scope : Scope
      settings: ActiveDisplayYMinimum=-3032.1328222995417  ActiveDisplayYMaximum=2924.7257482069263  DataLoggingVariableName=ScopeData21
  u1_dab_transformer : nesl_utility/PS-Simulink Converter  PhysicalDomain=network_engine_domain  SubClassName=ps_output  LeftPortType=input  RightPortType=output  PseudoPeriodic=off  Frequencies=[]  VectorFormat=1-D array  Unit=V  AffineConversion=on
  u2_dab_transformer : nesl_utility/PS-Simulink Converter  PhysicalDomain=network_engine_domain  SubClassName=ps_output  LeftPortType=input  RightPortType=output  PseudoPeriodic=off  Frequencies=[]  VectorFormat=1-D array  Unit=V  AffineConversion=on
  u1(+) : PMIOPort  Side=Left
  u2(+) : PMIOPort  Port=2  Side=Right
  u1(-) : PMIOPort  Port=3  Side=Left
  u2(-) : PMIOPort  Port=4  Side=Right
  tag scope: i1_dab_transformer_modA=global, i2_dab_transformer_modA=global, single_phase_transformer_data_modA=global, u1_dab_transformer_modA=global, u2_dab_transformer_modA=global
  wires:
  i2_dab_transformer/1 -> [i2_dab_transformer_modA]
  u2_dab_transformer/1 -> [u2_dab_transformer_modA]
  u1_dab_transformer/1 -> [u1_dab_transformer_modA]
  i1_dab_transformer/1 -> [i1_dab_transformer_modA]
  single_phase_transformer/1 -> [single_phase_transformer_data_modA], single_phase_transformer - scope/1
  connections:
  Current Sensor/RConn2 -- u2(+)/RConn1
  Voltage Sensor3/RConn2 -- single_phase_transformer/RConn2 -- u2(-)/RConn1
  Current Sensor/RConn1 -- i2_dab_transformer/LConn1
  Voltage Sensor3/RConn1 -- u2_dab_transformer/LConn1
  u1(-)/RConn1 -- single_phase_transformer/LConn2 -- Voltage Sensor1/RConn2
  Current Sensor1/LConn1 -- Voltage Sensor1/LConn1 -- u1(+)/RConn1
  Voltage Sensor1/RConn1 -- u1_dab_transformer/LConn1
  Current Sensor1/RConn1 -- i1_dab_transformer/LConn1
  Voltage Sensor3/LConn1 -- Capacitor1/RConn1 -- Current Sensor/LConn1
  single_phase_transformer/LConn1 -- Capacitor/RConn1
  single_phase_transformer/RConn1 -- Capacitor1/LConn1
  Capacitor/LConn1 -- Current Sensor1/RConn2
